simulink model "disturbance"  (R2026a)
settings: Solver=VariableStepAuto  StopTime=700
libraries: cstblocks_lti x4
settings Model: Creator=nelis  LastModifiedBy=nelis

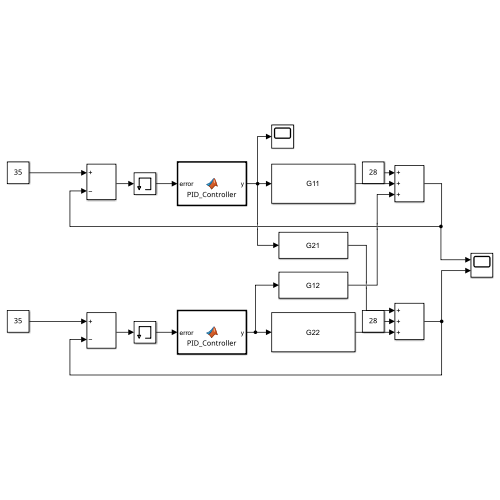
[thumbnail: Simulink's stored preview of the top-level diagram]
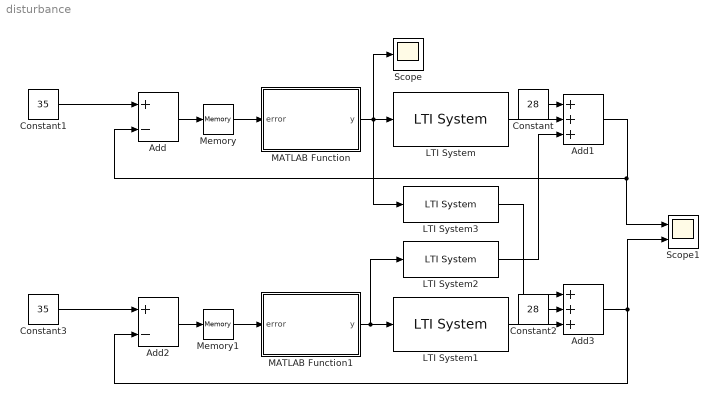
== system disturbance ==
  Add : Sum  Inputs=+-
  Add1 : Sum  Inputs=+++
  Add2 : Sum  Inputs=+-
  Add3 : Sum  Inputs=+++
  Constant : Constant  Value=28
  Constant1 : Constant  Value=35
  Constant2 : Constant  Value=28
  Constant3 : Constant  Value=35
  LTI System : cstblocks_lti/LTI System  sys=G11  IC=[]  PadeOrder=1
      settings: LibrarySourceBlock=cstblocks/LTI System
  LTI System1 : cstblocks_lti/LTI System  sys=G22  IC=[]  PadeOrder=1
      settings: LibrarySourceBlock=cstblocks/LTI System
  LTI System2 : cstblocks_lti/LTI System  sys=G12  IC=[]  PadeOrder=0
      settings: LibrarySourceBlock=cstblocks/LTI System
  LTI System3 : cstblocks_lti/LTI System  sys=G21  IC=[]  PadeOrder=0
      settings: LibrarySourceBlock=cstblocks/LTI System
  MATLAB Function : MATLAB Function  TreatAsAtomicUnit=on  SystemSampleTime=0.005
  MATLAB Function1 : MATLAB Function  TreatAsAtomicUnit=on  SystemSampleTime=0.005
  Memory : Memory
  Memory1 : Memory
  Scope : Scope
  Scope1 : Scope  NumInputPorts=2
      settings: ActiveDisplayYMinimum=26.957829925726386  ActiveDisplayYMaximum=37.379530668462536
  wires:
  Constant1/1 -> Add/1
  LTI System/1 -> Add1/2
  Add1/1 -> Scope1/1, Add/2
  Memory/1 -> MATLAB Function/1(error)
  Constant/1 -> Add1/1
  MATLAB Function/1(y) -> Scope/1, LTI System3/1, LTI System/1
  Add/1 -> Memory/1
  Constant3/1 -> Add2/1
  Constant2/1 -> Add3/2
  LTI System1/1 -> Add3/3
  MATLAB Function1/1(y) -> LTI System2/1, LTI System1/1
  Add3/1 -> Add2/2, Scope1/2
  Memory1/1 -> MATLAB Function1/1(error)
  Add2/1 -> Memory1/1
  LTI System2/1 -> Add1/3
  LTI System3/1 -> Add3/1

== matlab function disturbance/MATLAB Function ==
  data: y output; error input
function y =  PID_Controller(error)
    persistent prev_error;
    persistent integral;
    dt = 0.005;

    D = 1.1792;
    P = 0.1527141807;
    I = 0.00347932;

    if isempty(prev_error)
        prev_error = error;
    end

    if isempty(integral)
        integral = 0;
    end

    next_integral = integral + error * dt;
    derivative = (error - prev_error)/dt;

    pid_out = P*error + I*next_integral + D*derivative;

    if pid_out >= 3.3
        pid_out = 3.3;
        if error < 0
            integral = next_integral;
        end

    elseif pid_out < 0
        pid_out = 0;
        if error > 0
            integral = next_integral;
        end
    else
        integral = next_integral;
    end

    prev_error = error;

y = pid_out;

== matlab function disturbance/MATLAB Function1 ==
  data: y output; error input
function y =  PID_Controller(error)
    persistent prev_error;
    persistent integral;
    dt = 0.005;

    D = 1.906;
    P = 0.2328623;
    I = 0.00422623;

    if isempty(prev_error)
        prev_error = error;
    end

    if isempty(integral)
        integral = 0;
    end

    next_integral = integral + error * dt;
    derivative = (error - prev_error)/dt;

    pid_out = P*error + I*next_integral + D*derivative;

    if pid_out >= 3.3
        pid_out = 3.3;
        if error < 0
            integral = next_integral;
        end

    elseif pid_out < 0
        pid_out = 0;
        if error > 0
            integral = next_integral;
        end
    else
        integral = next_integral;
    end

    prev_error = error;

y = pid_out;
